simulink model "NLMS_Sec_path_est"  (R2023a)
settings: Solver=ode1be  StartTime=0.0  StopTime=40.0  FixedStep=Ts  RelTol=1e-3
values from neighbouring files (symbols this model uses):
  L = 200    [Initialization_1x1x1.m]    (also in Initialization_1x2x2.m = 100; Initialization_fxKalman.m = 70; Initialization_path_estimation.m = 100)
  Ts = 1/fs    (= 0.001)    [Initialization_1x1x1.m]    (also in Initialization_1x2x2.m; Initialization_fxKalman.m; Initialization_path_estimation.m)
libraries: speedgoatlib_IO104 x3, dspsrcs4 x1, dspadpt3 x1
settings Model: Creator=Tamida  LastModifiedBy=tislam
settings SolverCC: ConcurrentTasks=on  PositivePriorityOrder=on
settings DataIOCC: LimitDataPoints=on  MaxDataPoints=1  SaveOutput=off  SignalLogging=off  DSMLogging=off  SaveTime=off  ReturnWorkspaceOutputs=off
settings OptimizationCC: BlockReduction=off  OptimizeBlockIOStorage=off  ReuseModelBlockBuffer=off
settings DebuggingCC: TasksWithSamePriorityMsg=none
settings HardwareCC: ProdBitPerLong=64  ProdLongLongMode=on  ProdHWDeviceType=Intel->x86-64 (Linux 64)
settings RTWCC: Description=Simulink Real-Time  SystemTargetFile=slrealtime.tlc  TemplateMakefile=slrealtime_default_tmf  Toolchain=Simulink Real-Time Toolchain  BuildConfiguration=Faster Runs  CodeExecutionProfiling=on  TargetLang=C++

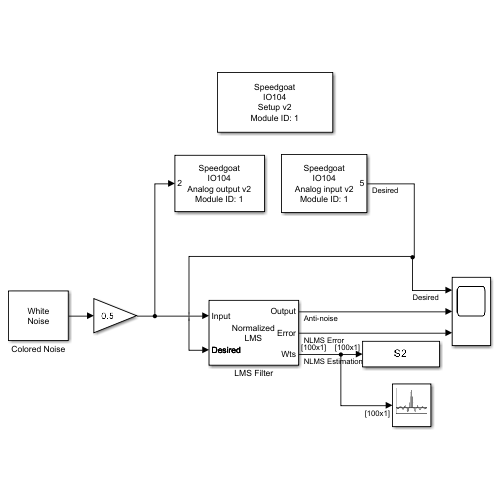
[thumbnail: Simulink's stored preview of the top-level diagram]
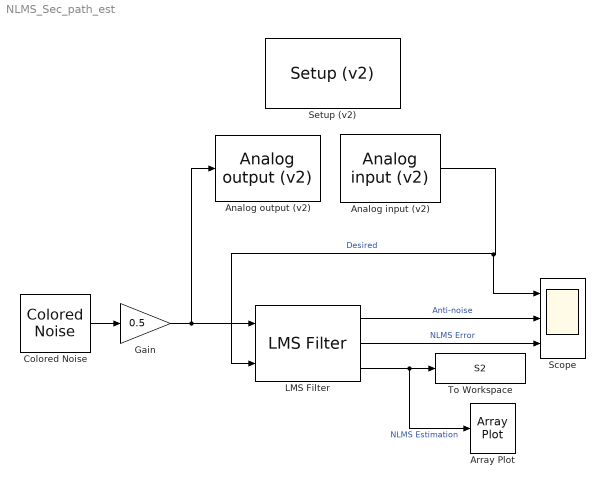
== system NLMS_Sec_path_est ==
  "Analog input (v2) " : speedgoatlib_IO104/Analog input (v2)   parModuleId=1  parTs=Ts  parPciSlot=-1  parAdChannels=5  parAdChannelsSorted=5  parAdRange1=+-2.5V  parAdRange2=+-2.5V  parAdCoupling=Differential  parAdFrameSize=1  parAdUseTrigger=off  parAdClockInitiator=Initiator  parAdSampleTime=1.000000000e-03  parTriggerInitiator=Initiator  parTriggerRate=-1.000000000e+00
      settings: SourceProductName=Simulink Real-Time: Speedgoat I/O Blockset
  "Analog output (v2) " : speedgoatlib_IO104/Analog output (v2)   parModuleId=1  parTs=Ts  parPciSlot=-1  parDaSimultaneous=on  parDaChannels=2  parDaChannelsSorted=2  parDaInitValue=0  parDaReset=1  parDaRange=+-2.5V  parDaFrameSize=1  parDaUseTrigger=off  parDaClockInitiator=Initiator  parDaSampleTime=1.000000000e-03  parTriggerInitiator=Initiator  parTriggerRate=-1.000000000e+00  parAdBlockPresent=1
      settings: SourceProductName=Simulink Real-Time: Speedgoat I/O Blockset
  Array Plot : ArrayPlot  WindowPosition=[8.000000,48.000000,1265.000000,643.000000,]  ScopeFrameLocation=window  YLimits=[-0.7629,0.7053]
  Colored Noise : dspsrcs4/Colored Noise  Color=white  InverseFrequencyPower=1  BoundedOutput=on  NumChannels=1  OutputDataType=double  SamplesPerFrame=1  SampleTime=Ts  RandomStream=mt19937ar with seed  Seed=67  SimulateUsing=Interpreted execution
      settings: LibrarySourceBlock=audiosources/Colored Noise
  Gain : Gain  Gain=0.5
  LMS Filter : dspadpt3/LMS Filter  Algo=Normalized LMS  L=L  stepflag=Dialog  mu=0.05  leakage=1  ic=0  Adapt=off  resetflag=None  weights=on  addnparflag=off  roundingMode=Floor  overflowMode=off  secondCoeffMode=Binary point scaling  secondCoeffWordLength=2  secondCoeffFracLength=15  memoryMode=Binary point scaling  memoryWordLength=16  memoryFracLength=15  prodOutput2Mode=Binary point scaling  prodOutput2FracLength=20  prodOutput3Mode=Binary point scaling  prodOutput3FracLength=20  prodOutput4Mode=Binary point scaling  prodOutput4FracLength=20  quotientMode=Binary point scaling  quotientFracLength=20  accum2Mode=Binary point scaling  accum2FracLength=20
      settings: LibrarySourceBlock=dsphdlsupportfiltering/LMS Filter
  Scope : Scope  NumInputPorts=3
  "Setup (v2) " : speedgoatlib_IO104/Setup (v2)   parPciSlot=-1  parModuleId=1  parTriggerInitiator=Initiator  parTriggerRate=Ts  parCalibrate=on  parAdChannels=[5]  parAdRange1=+-2.5V  parAdRange2=+-2.5V  parAdCoupling=Differential  parAdUseTrigger=off  parAdFrameSize=1  parAdClockInitiator=Initiator  parAdSampleTime=Ts  parDaSimultaneous=on  parDaChannels=[2]  parDaChannelsSorted=2  parDaInitValue=[0]  parDaReset=[1]  parDaRange=+-2.5V  parDaUseTrigger=off  parDaFrameSize=1  parDaClockInitiator=Initiator  parDaSampleTime=Ts  parDioByte0Dir=Outputs  parDioByte1Dir=Inputs  parDoChannels=[1]  parDoInitValues=[0]  parDoReset=[1]  parDiChannels=[1]
      settings: SourceProductName=Simulink Real-Time: Speedgoat I/O Blockset
  To Workspace : ToWorkspace  VariableName=S2  SampleTime=Ts
      settings: MaxDataPoints=L  Save2DSignal=2-D array (concatenate along first dimension)
  wires:
  "Analog input (v2) "/1 -> LMS Filter/2, Scope/1  "Desired"
  LMS Filter/2 -> Scope/3  "NLMS Error"
  LMS Filter/3 -> Array Plot/1, To Workspace/1  "NLMS Estimation"
  Colored Noise/1 -> Gain/1
  LMS Filter/1 -> Scope/2  "Anti-noise"
  Gain/1 -> LMS Filter/1, "Analog output (v2) "/1
